simulink model "SupervisorFSM_RX"  (R2023b)
settings: Solver=FixedStepDiscrete  StartTime=0.0  StopTime=10.0  FixedStep=Ts_SupervisorFSM_RX  RelTol=1e-3  EnableMultiTasking=on
undefined symbols (not defined in the file): InitConfParams
settings Model: DataDictionary=EmbeddedBoardDD.sldd  Creator=vvasco  LastModifiedBy=upattacini
settings SolverCC: AllowMultiTaskInputOutput=on  AlgebraicLoopSolver=TrustRegion  AutoInsertRateTranBlk=on  InsertRTBMode=Never (minimum delay)
settings DataIOCC: LimitDataPoints=on  SaveOutput=off  SignalLogging=off  DSMLogging=off  SaveTime=off  ReturnWorkspaceOutputs=off
settings OptimizationCC: DefaultParameterBehavior=Inlined  DefaultUnderspecifiedDataType=single  StrengthReduction=on  PassReuseOutputArgsAs=Individual arguments  ZeroExternalMemoryAtStartup=off  ZeroInternalMemoryAtStartup=off  OptimizeBlockOrder=speed  OptimizationPriority=Speed  OptimizationCustomize=off  MultiThreadedLoops=on  EfficientTunableParamExpr=on
settings DebuggingCC: ParameterPrecisionLossMsg=none  UnconnectedInputMsg=warning  UnconnectedOutputMsg=warning  UnconnectedLineMsg=warning  AllowSymbolicDim=off  SFUnexpectedBacktrackingDiag=warning  SFNoUnconditionalDefaultTransitionDiag=warning  SFExecutionAtInitializationDiag=none  ArithmeticOperatorsInVariantConditions=warning
settings HardwareCC: ProdBitPerPointer=32  ProdBitPerSizeT=32  ProdBitPerPtrDiffT=32  ProdLargestAtomicInteger=Long  ProdLargestAtomicFloat=Double  ProdWordSize=32  ProdHWDeviceType=ARM Compatible->ARM Cortex-M
settings ModelReferenceCC: UpdateModelReferenceTargets=Force  EnableRefExpFcnMdlSchedulingChecks=on  ModelReferenceNumInstancesAllowed=Single
settings SFSimCC: SimUseLocalCustomCode=off  MATLABDynamicMemAlloc=off  CustomCodeUndefinedFunction=UseInterfaceOnly
settings SFSimCC: SimCustomHeaderCode=|
  | #include "rtw_enable_disable_motors.h"
  | #include "rtw_motor_config.h"
settings SFSimCC: SimUserSources=|
  | rtw_enable_disable_motors.c
  | rtw_motor_config.c
settings RTWCC: Description=Embedded Coder  SystemTargetFile=ert.tlc  GenCodeOnly=on  PackageGeneratedCodeAndArtifacts=on  PackageName=SupervisorFSM_RX  TemplateMakefile=ert_default_tmf  GenerateReport=on  RTWUseLocalCustomCode=off  RTWUseSimCustomCode=on  LaunchReport=on  TargetLang=C++  GenerateCodeReplacementReport=on  DLArmComputeVersion=19.05
settings RTWCC: CustomHeaderCode=|
  | #include "rtw_enable_disable_motors.h"
  | #include "rtw_motor_config.h"
settings RTWCC: CustomSource=|
  | rtw_enable_disable_motors.c
  | rtw_motor_config.c
settings CodeAppCC: ForceParamTrailComments=on  IgnoreCustomStorageClasses=off  MaxIdLength=60  OperatorAnnotations=on  SimulinkDataObjDesc=on  SFDataObjDesc=on  InsertBlockDesc=on
settings ERTTargetCC: TargetLangStandard=C++03 (ISO)  CodeReplacementLibrary=ARM Cortex-M,iCubTech  GenerateSampleERTMain=on  SupportVariableSizeSignals=on  InlinedParameterPlacement=NonHierarchical  RootIOFormat=Structure reference  ERTCustomFileTemplate=example_file_process.tlc
settings ConfigComp: CovMetricSettings=dw  CovSaveCumulativeToWorkspaceVar=on  CovSaveSingleToWorkspaceVar=on  CovExternalEMLEnable=off

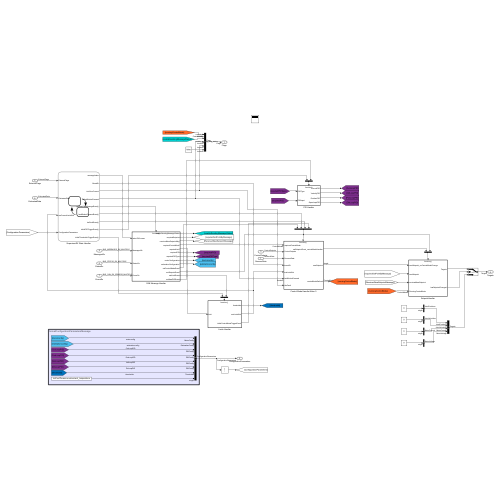
[thumbnail: Simulink's stored preview of the top-level diagram]
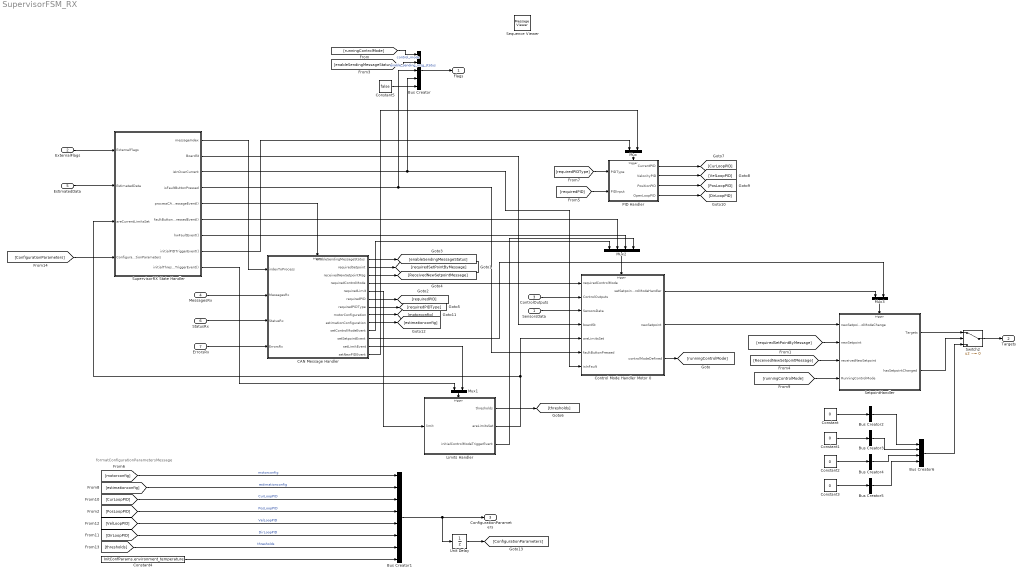
== system SupervisorFSM_RX ==
  note: formatConfigurationParametersMessage
  SensorsData : Inport  OutDataTypeStr=Bus: SensorsData  BusOutputAsStruct=on
  ExternalFlags : Inport  Port=2  OutDataTypeStr=Bus: ExternalFlags  BusOutputAsStruct=on
  ControlOutputs : Inport  Port=3  OutDataTypeStr=Bus: ControlOutputs  BusOutputAsStruct=on
  MessagesRx : Inport  Port=4  OutDataTypeStr=Bus: BUS_MESSAGES_RX_MULTIPLE  BusOutputAsStruct=on
  EstimatedData : Inport  Port=5  OutDataTypeStr=Bus: EstimatedData  BusOutputAsStruct=on
  StatusRx : Inport  Port=6  OutDataTypeStr=Bus: BUS_STATUS_RX_MULTIPLE  BusOutputAsStruct=on
  ErrorsRx : Inport  Port=7  OutDataTypeStr=Bus: BUS_CAN_RX_ERRORS_MULTIPLE  BusOutputAsStruct=on
  Bus Creator : BusCreator  Inputs=5  OutDataTypeStr=Bus: Flags  NonVirtualBus=on
      settings: InheritFromInputs=off
  Bus Creator1 : BusCreator  Inputs=8  OutDataTypeStr=Bus: ConfigurationParameters  NonVirtualBus=on
      settings: InheritFromInputs=off
  Bus Creator2 : BusCreator  Inputs=1  OutDataTypeStr=Bus: JointPositions  NonVirtualBus=on
      settings: InheritFromInputs=off
  Bus Creator3 : BusCreator  Inputs=1  OutDataTypeStr=Bus: JointVelocities  NonVirtualBus=on
      settings: InheritFromInputs=off
  Bus Creator4 : BusCreator  Inputs=1  OutDataTypeStr=Bus: MotorCurrent  NonVirtualBus=on
      settings: InheritFromInputs=off
  Bus Creator5 : BusCreator  Inputs=1  OutDataTypeStr=Bus: MotorVoltage  NonVirtualBus=on
      settings: InheritFromInputs=off
  Bus Creator6 : BusCreator  Inputs=4  OutDataTypeStr=Bus: Targets  NonVirtualBus=on
      settings: InheritFromInputs=off
  CAN Message Handler : Subsystem
  Constant{,1..3} (4 alike) : Constant  Value=0  OutDataTypeStr=single
  Constant4 : Constant  Value=InitConfParams.environment_temperature
  Constant5 : Constant  Value=false  OutDataTypeStr=boolean
  Control Mode Handler Motor 0 : Subsystem  TreatAsAtomicUnit=on
  Limits Handler : Subsystem  TreatAsAtomicUnit=on
  Mux : Mux  Inputs=2
  Mux1 : Mux  Inputs=2
  Mux2 : Mux
  Mux3 : Mux  Inputs=2
  PID Handler : Subsystem
  Sequence Viewer : MessageViewer  History=1000  SavedRootId=#
  SetpointHandler : Subsystem  TreatAsAtomicUnit=on
  SupervisorRX State Handler : Stateflow chart  TreatAsAtomicUnit=on
  Switch2 : Switch  Criteria=u2 ~= 0  SaturateOnIntegerOverflow=off  InputSameDT=off
  Unit Delay : UnitDelay  SampleTime=-1  HasFrameUpgradeWarning=on
  Flags : Outport  OutDataTypeStr=Bus: Flags  BusOutputAsStruct=on
  Targets : Outport  Port=2  OutDataTypeStr=Bus: Targets  BusOutputAsStruct=on
  ConfigurationParameters : Outport  Port=3  OutDataTypeStr=Bus: ConfigurationParameters  BusOutputAsStruct=on
  wires:
  ControlOutputs/1 -> Control Mode Handler Motor 0/2(ControlOutputs)
  ExternalFlags/1 -> SupervisorRX State Handler/1(ExternalFlags)
  SupervisorRX State Handler/1(messageIndex) -> CAN Message Handler/1(indexToProcess)
  SupervisorRX State Handler/2(BoardSt) -> Control Mode Handler Motor 0/4(boardSt)
  SupervisorRX State Handler/3(isInOverCurrent) -> Control Mode Handler Motor 0/7(isInFault), Bus Creator/4
  SupervisorRX State Handler/5(processCANMessageEvent()) -> CAN Message Handler/Trigger
  StatusRx/1 -> CAN Message Handler/3(StatusRx)
  MessagesRx/1 -> CAN Message Handler/2(MessagesRx)
  ErrorsRx/1 -> CAN Message Handler/4(ErrorsRx)
  CAN Message Handler/1(enableSendingMessageStatus) -> [enableSendingMessageStatus]
  CAN Message Handler/2(requiredSetpoint) -> [requiredSetPointByMessage]
  CAN Message Handler/4(requiredControlMode) -> Control Mode Handler Motor 0/1(requiredControlMode)
  CAN Message Handler/11(setSetpointEvent) -> Mux3/2
  CAN Message Handler/12(setLimitEvent) -> Mux1/2
  CAN Message Handler/5(requiredLimit) -> Limits Handler/1(limit)
  CAN Message Handler/10(setControlModeEvent) -> Mux2/1
  Limits Handler/1(thresholds) -> [thresholds]
  Limits Handler/2(areLimitsSet) -> Control Mode Handler Motor 0/5(areLimitsSet), SupervisorRX State Handler/3(areCurrentLimitsSet)
  SensorsData/1 -> Control Mode Handler Motor 0/3(SensorsData)
  SupervisorRX State Handler/4(isFaultButtonPressed) -> Control Mode Handler Motor 0/6(faultButtonPressed), Bus Creator/3
  Control Mode Handler Motor 0/1(setSetpointEvent_controlModeHandler) -> Mux3/1
  Control Mode Handler Motor 0/3(controlModeDefined) -> [runningControlMode]
  Control Mode Handler Motor 0/2(newSetpoint) -> SetpointHandler/1(newSetpoint_onControlModeChange)
  SupervisorRX State Handler/6(faultButtonPressedEvent()) -> Mux2/2
  SupervisorRX State Handler/7(hwFaultEvent()) -> Mux2/3
  Mux2/1 -> Control Mode Handler Motor 0/Trigger
  [runningControlMode] -> Bus Creator/1  "control_mode"
  [enableSendingMessageStatus] -> Bus Creator/2  "enable_sending_msg_status"
  Bus Creator/1 -> Flags/1
  [requiredSetPointByMessage] -> SetpointHandler/2(newSetpoint)
  SetpointHandler/2(hasSetpointChanged) -> Switch2/2
  Switch2/1 -> Targets/1
  SetpointHandler/1(Targets) -> Switch2/1
  Bus Creator2/1 -> Bus Creator6/1
  Constant3/1 -> Bus Creator5/1
  Bus Creator3/1 -> Bus Creator6/2
  Bus Creator5/1 -> Bus Creator6/4
  Bus Creator4/1 -> Bus Creator6/3
  Constant2/1 -> Bus Creator4/1
  Constant1/1 -> Bus Creator3/1
  Constant/1 -> Bus Creator2/1
  Bus Creator6/1 -> Switch2/3
  Bus Creator1/1 -> ConfigurationParameters/1, Unit Delay/1
  Mux3/1 -> SetpointHandler/Trigger
  CAN Message Handler/3(receivedNewSetpointMsg) -> [ReceivedNewSetpointMessage]
  [ReceivedNewSetpointMessage] -> SetpointHandler/3(receivedNewSetpoint)
  [runningControlMode] -> SetpointHandler/4(RunningControlMode)
  Limits Handler/3(initialControlModeTriggerEvent) -> Mux2/4
  CAN Message Handler/13(setNewPIDEvent) -> Mux/2
  CAN Message Handler/6(requiredPID) -> [requiredPID]
  CAN Message Handler/7(requiredPIDType) -> [requiredPIDType]
  [requiredPIDType] -> PID Handler/1(PIDType)
  [requiredPID] -> PID Handler/2(PIDInput)
  PID Handler/1(CurrentPID) -> [CurLoopPID]
  PID Handler/2(VelocityPID) -> [VelLoopPID]
  PID Handler/3(PositionPID) -> [PosLoopPID]
  PID Handler/4(OpenLoopPID) -> [DirLoopPID]
  CAN Message Handler/8(motorConfiguration) -> [motorconfig]
  CAN Message Handler/9(estimationConfiguration) -> [estimationconfig]
  [PosLoopPID] -> Bus Creator1/4  "PosLoopPID"
  [VelLoopPID] -> Bus Creator1/5  "VelLoopPID"
  [DirLoopPID] -> Bus Creator1/6  "DirLoopPID"
  [CurLoopPID] -> Bus Creator1/3  "CurLoopPID"
  [motorconfig] -> Bus Creator1/1  "motorconfig"
  [estimationconfig] -> Bus Creator1/2  "estimationconfig"
  [thresholds] -> Bus Creator1/7  "thresholds"
  Unit Delay/1 -> [ConfigurationParameters]
  [ConfigurationParameters] -> SupervisorRX State Handler/4(ConfigurationParameters)
  Mux/1 -> PID Handler/Trigger
  Mux1/1 -> Limits Handler/Trigger
  SupervisorRX State Handler/8(initialPIDTriggerEvent()) -> Mux/1
  SupervisorRX State Handler/9(initialThresholdsTriggerEvent()) -> Mux1/1
  EstimatedData/1 -> SupervisorRX State Handler/2(EstimatedData)
  Constant4/1 -> Bus Creator1/8
  Constant5/1 -> Bus Creator/5

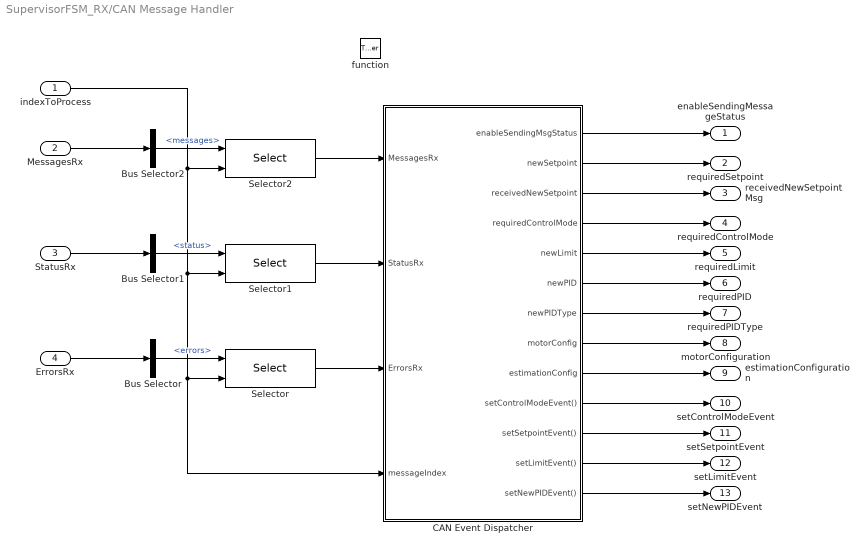
== system SupervisorFSM_RX/CAN Message Handler ==
  indexToProcess : Inport
  MessagesRx : Inport  Port=2  OutDataTypeStr=Bus: BUS_MESSAGES_RX_MULTIPLE
  StatusRx : Inport  Port=3  OutDataTypeStr=Bus: BUS_STATUS_RX_MULTIPLE
  ErrorsRx : Inport  Port=4  OutDataTypeStr=Bus: BUS_CAN_RX_ERRORS_MULTIPLE
  function : TriggerPort  TriggerType=function-call  VariantControl=(inherit)
  Bus Selector : BusSelector  OutputSignals=errors
  Bus Selector1 : BusSelector  OutputSignals=status
  Bus Selector2 : BusSelector  OutputSignals=messages
  CAN Event Dispatcher : Stateflow chart  TreatAsAtomicUnit=on
      settings: PortSchema="{\"entries\":[{\"content\":{\"sides\":[{\"content\":{\"connectorIds\":[\"In3\",\"In2\",\"In1\",\"In4\"]},\"type\":\"ConnectorPlacement.EquallySpacedRectSide\",\"uuid\":\"262d8322-eee9-4d2f-8394-9ad0f57315f2\"},{\"content\":{\"connectorIds\":[\"Out4\",\"Out2\",\"Out5\",\"Out1\",\"Out3\",\"Out6\",\"Out7\",\"Out8\",\"Out9\",\"Out10\",\"Out11\",\"Out12\",\"Out13\"],\"side\":\"RIGHT\"},\"type\":\"ConnectorPlacement.EquallySpacedRectSide\",\"uuid\":\"ca9d82ac-748f-4018-bf9f-4633821aba3f\"},{\"content\":{\"connectorIds\":[],\"side\":\"TOP\"},\"type\":\"ConnectorPlacement.EquallySpacedRectSide\",\"uuid\":\"6799758e-9858-4ae3-a4b1-29346dfc98be\"}]},\"type\":\"ConnectorPlacement.EquallySpacedConnector\",\"uuid\":\"ac16e6b5-85f8-470c-98ca-7de9ad02246e\"}],\"packageUris\":[\"http://schema.mathworks.com/mf0/Connector/R2020b\"],\"version\":\"1.0\"}"
  Selector : Selector  NumberOfDimensions=2  InputPortWidth=3  IndexOptions=Index vector (dialog),Index vector (port)  Indices=1,1  OutputSizes=1,1
  Selector1 : Selector  NumberOfDimensions=2  InputPortWidth=3  IndexOptions=Index vector (dialog),Index vector (port)  Indices=1,1  OutputSizes=1,1
  Selector2 : Selector  NumberOfDimensions=2  InputPortWidth=3  IndexOptions=Index vector (dialog),Index vector (port)  Indices=1,1  OutputSizes=1,1
  enableSendingMessageStatus : Outport
  requiredSetpoint : Outport  Port=2
  receivedNewSetpointMsg : Outport  Port=3
  requiredControlMode : Outport  Port=4
  requiredLimit : Outport  Port=5
  requiredPID : Outport  Port=6  OutDataTypeStr=Bus: BUS_MSG_PID
  requiredPIDType : Outport  Port=7
  motorConfiguration : Outport  Port=8  OutDataTypeStr=Bus: MotorConfig
  estimationConfiguration : Outport  Port=9  OutDataTypeStr=Bus: EstimationConfig
  setControlModeEvent : Outport  Port=10
  setSetpointEvent : Outport  Port=11
  setLimitEvent : Outport  Port=12
  setNewPIDEvent : Outport  Port=13
  wires:
  ErrorsRx/1 -> Bus Selector/1
  StatusRx/1 -> Bus Selector1/1
  MessagesRx/1 -> Bus Selector2/1
  Bus Selector2/1 -> Selector2/1  "<messages>"
  Bus Selector1/1 -> Selector1/1  "<status>"
  Bus Selector/1 -> Selector/1  "<errors>"
  indexToProcess/1 -> Selector1/2, CAN Event Dispatcher/4(messageIndex), Selector/2, Selector2/2
  Selector/1 -> CAN Event Dispatcher/1(ErrorsRx)
  Selector1/1 -> CAN Event Dispatcher/2(StatusRx)
  Selector2/1 -> CAN Event Dispatcher/3(MessagesRx)
  CAN Event Dispatcher/1(requiredControlMode) -> requiredControlMode/1
  CAN Event Dispatcher/10(setControlModeEvent()) -> setControlModeEvent/1
  CAN Event Dispatcher/11(setSetpointEvent()) -> setSetpointEvent/1
  CAN Event Dispatcher/12(setLimitEvent()) -> setLimitEvent/1
  CAN Event Dispatcher/4(enableSendingMsgStatus) -> enableSendingMessageStatus/1
  CAN Event Dispatcher/2(newSetpoint) -> requiredSetpoint/1
  CAN Event Dispatcher/3(newLimit) -> requiredLimit/1
  CAN Event Dispatcher/5(receivedNewSetpoint) -> receivedNewSetpointMsg/1
  CAN Event Dispatcher/6(newPID) -> requiredPID/1
  CAN Event Dispatcher/7(newPIDType) -> requiredPIDType/1
  CAN Event Dispatcher/8(motorConfig) -> motorConfiguration/1
  CAN Event Dispatcher/13(setNewPIDEvent()) -> setNewPIDEvent/1
  CAN Event Dispatcher/9(estimationConfig) -> estimationConfiguration/1

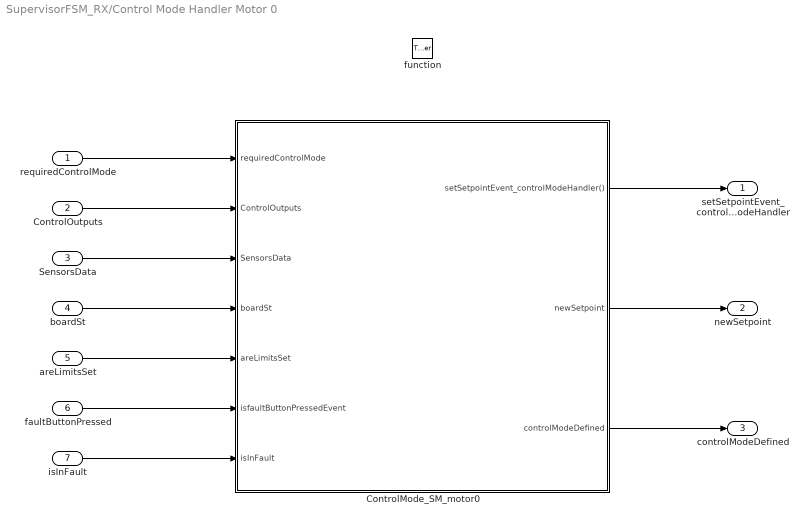
== system SupervisorFSM_RX/Control Mode Handler Motor 0 ==
  requiredControlMode : Inport  OutDataTypeStr=Enum: ControlModes
  ControlOutputs : Inport  Port=2  OutDataTypeStr=Bus: ControlOutputs
  SensorsData : Inport  Port=3  OutDataTypeStr=Bus: SensorsData
  boardSt : Inport  Port=4
  areLimitsSet : Inport  Port=5
  faultButtonPressed : Inport  Port=6  OutDataTypeStr=boolean
  isInFault : Inport  Port=7
  function : TriggerPort  TriggerType=function-call  VariantControl=(inherit)  OutputDataType=double
  ControlMode_SM_motor0 : Stateflow chart  TreatAsAtomicUnit=on
      settings: PortSchema="{\"entries\":[{\"content\":{\"sides\":[{\"content\":{\"connectorIds\":[\"In3\",\"In5\",\"In4\",\"In1\",\"In2\",\"In6\",\"In7\"]},\"type\":\"ConnectorPlacement.EquallySpacedRectSide\",\"uuid\":\"16512c25-bd76-4850-9767-5b856cef53aa\"},{\"content\":{\"connectorIds\":[\"Out3\",\"Out1\",\"Out2\"],\"side\":\"RIGHT\"},\"type\":\"ConnectorPlacement.EquallySpacedRectSide\",\"uuid\":\"18a45251-a2e9-43d4-bd88-b12ad9528921\"},{\"content\":{\"connectorIds\":[],\"side\":\"TOP\"},\"type\":\"ConnectorPlacement.EquallySpacedRectSide\",\"uuid\":\"fd5907c5-7215-4be4-b0f8-eb015da6c502\"}]},\"type\":\"ConnectorPlacement.EquallySpacedConnector\",\"uuid\":\"dd0cc5ef-a33e-40fc-9b84-b3bdf02167fe\"}],\"packageUris\":[\"http://schema.mathworks.com/mf0/Connector/R2020b\"],\"version\":\"1.0\"}"
  setSetpointEvent_controlModeHandler : Outport
  newSetpoint : Outport  Port=2  OutDataTypeStr=single
  controlModeDefined : Outport  Port=3  OutDataTypeStr=Enum: ControlModes
  wires:
  boardSt/1 -> ControlMode_SM_motor0/1(boardSt)
  areLimitsSet/1 -> ControlMode_SM_motor0/2(areLimitsSet)
  requiredControlMode/1 -> ControlMode_SM_motor0/3(requiredControlMode)
  SensorsData/1 -> ControlMode_SM_motor0/4(SensorsData)
  ControlOutputs/1 -> ControlMode_SM_motor0/5(ControlOutputs)
  ControlMode_SM_motor0/2(controlModeDefined) -> controlModeDefined/1
  ControlMode_SM_motor0/1(newSetpoint) -> newSetpoint/1
  ControlMode_SM_motor0/3(setSetpointEvent_controlModeHandler()) -> setSetpointEvent_controlModeHandler/1
  faultButtonPressed/1 -> ControlMode_SM_motor0/6(isfaultButtonPressedEvent)
  isInFault/1 -> ControlMode_SM_motor0/7(isInFault)

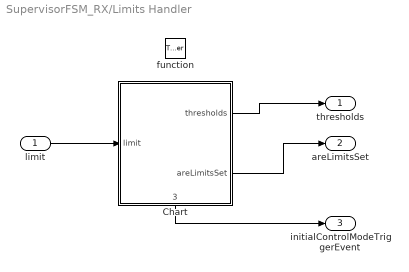
== system SupervisorFSM_RX/Limits Handler ==
  limit : Inport
  function : TriggerPort  TriggerType=function-call  VariantControl=(inherit)
  Chart : Stateflow chart  TreatAsAtomicUnit=on
      settings: PortSchema="{\"entries\":[{\"content\":{\"sides\":[{\"content\":{\"connectorIds\":[\"In1\"]},\"type\":\"ConnectorPlacement.EquallySpacedRectSide\",\"uuid\":\"0584a8d9-54fc-4826-bb82-8ee436931ccb\"},{\"content\":{\"connectorIds\":[\"Out1\",\"Out2\"],\"side\":\"RIGHT\"},\"type\":\"ConnectorPlacement.EquallySpacedRectSide\",\"uuid\":\"1e00f1d2-76af-45ba-9501-0555e9c73a7d\"},{\"content\":{\"connectorIds\":[],\"side\":\"TOP\"},\"type\":\"ConnectorPlacement.EquallySpacedRectSide\",\"uuid\":\"c8be2aa1-781d-4a54-8da4-289e5dceeb67\"},{\"content\":{\"connectorIds\":[\"Out3\"],\"side\":\"BOTTOM\"},\"type\":\"ConnectorPlacement.EquallySpacedRectSide\",\"uuid\":\"c0009a38-640d-457e-891e-a241b21e5d3e\"}]},\"type\":\"ConnectorPlacement.EquallySpacedConnector\",\"uuid\":\"a709c32b-ef0c-4b14-b7ff-ec32eaa315cd\"}],\"packageUris\":[\"http://schema.mathworks.com/mf0/Connector/R2020b\"],\"version\":\"1.0\"}"
  thresholds : Outport
  areLimitsSet : Outport  Port=2
  initialControlModeTriggerEvent : Outport  Port=3
  wires:
  Chart/1(thresholds) -> thresholds/1
  Chart/2(areLimitsSet) -> areLimitsSet/1
  limit/1 -> Chart/1(limit)
  Chart/3(initialControlModeTriggerEvent()) -> initialControlModeTriggerEvent/1

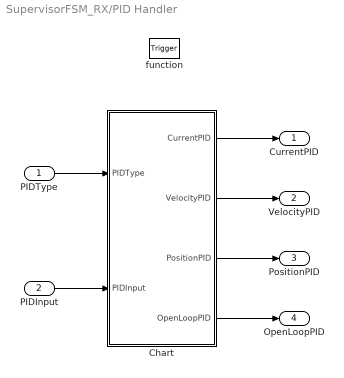
== system SupervisorFSM_RX/PID Handler ==
  PIDType : Inport
  PIDInput : Inport  Port=2
  function : TriggerPort  TriggerType=function-call  VariantControl=(inherit)
  Chart : Stateflow chart  TreatAsAtomicUnit=on
  CurrentPID : Outport
  VelocityPID : Outport  Port=2
  PositionPID : Outport  Port=3
  OpenLoopPID : Outport  Port=4
  wires:
  PIDType/1 -> Chart/1(PIDType)
  PIDInput/1 -> Chart/2(PIDInput)
  Chart/2(VelocityPID) -> VelocityPID/1
  Chart/3(PositionPID) -> PositionPID/1
  Chart/4(OpenLoopPID) -> OpenLoopPID/1
  Chart/1(CurrentPID) -> CurrentPID/1

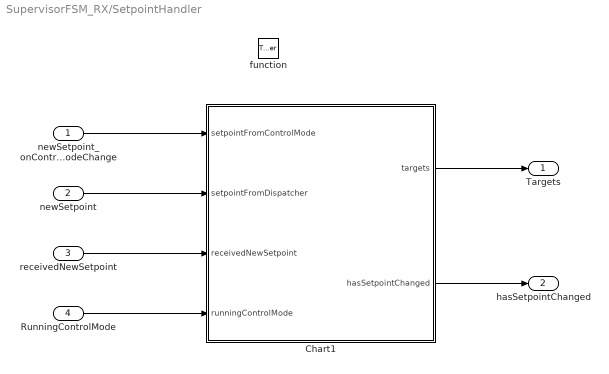
== system SupervisorFSM_RX/SetpointHandler ==
  newSetpoint_onControlModeChange : Inport
  newSetpoint : Inport  Port=2
  receivedNewSetpoint : Inport  Port=3
  RunningControlMode : Inport  Port=4  OutDataTypeStr=Enum: ControlModes
  function : TriggerPort  TriggerType=function-call  VariantControl=(inherit)
  Chart1 : Stateflow chart  TreatAsAtomicUnit=on
  Targets : Outport  OutDataTypeStr=Bus: Targets
  hasSetpointChanged : Outport  Port=2
  wires:
  newSetpoint_onControlModeChange/1 -> Chart1/1(setpointFromControlMode)
  newSetpoint/1 -> Chart1/2(setpointFromDispatcher)
  Chart1/2(hasSetpointChanged) -> hasSetpointChanged/1
  Chart1/1(targets) -> Targets/1
  receivedNewSetpoint/1 -> Chart1/3(receivedNewSetpoint)
  RunningControlMode/1 -> Chart1/4(runningControlMode)

== stateflow chart SupervisorFSM_RX/Limits Handler/Chart ==
  state Home
  (junction 31) -> (junction 33)
  (junction 11) -> (junction 31) [order 1] : [areLimitsSet == false]
      | {areLimitsSet = true;
      | send(initialControlModeTriggerEvent);}
  (junction 33) -> (junction 21)
  (junction 11) -> (junction 21) [order 2]
  (junction 2) -> (junction 11) [order 1] : [limit.type == ControlModes.Current]
      | {thresholds.motorNominalCurrents = abs(limit.nominal);
      | thresholds.motorPeakCurrents = abs(limit.peak);
      | thresholds.motorOverloadCurrents = abs(limit.overload);}
  (junction 21) -> Home
  (default) -> (junction 2) : {thresholds=InitConfParams.thresholds;}
  Home -> (junction 2)
  (junction 2) -> (junction 16) [order 2]
  (junction 25) -> Home
  (junction 16) -> (junction 25)
  data: thresholds output Bus: Thresholds; areLimitsSet output boolean =false; limit input Bus: SV_Limits; InitConfParams parameter Bus: ConfigurationParameters
  events: initialControlModeTriggerEvent output FUNCTION_CALL_EVENT

== stateflow chart SupervisorFSM_RX/SupervisorRX State Handler ==
  state STATE_HANDLER [parallel]
    settings: executionOrder=1
    note: ATTENTION :
        | Currently the events "BoardFaultEvent" and "OutOfBoardFaultEvent"
        | are not sent by any state. They are simple placeholder.
    state NotConfigured
      entry:
      BoardSt = BoardState.NotConfigured;
    state Fault
      entry:
      BoardSt = BoardState.Fault;
    state Configured
      entry:
      BoardSt = BoardState.Configured;
    (default) -> NotConfigured
    NotConfigured -> Fault [order 1] : BoardFaultEvent
    (junction 548) -> NotConfigured [order 1] : [!isBoardConfigured()]
    NotConfigured -> Configured [order 2] : [isBoardConfigured()]
    (junction 548) -> Configured [order 2]
    Fault -> (junction 548) : OutOfBoardFaultEvent
    Configured -> Fault : BoardFaultEvent
  state FAULT_HANDLER [parallel]
    settings: executionOrder=2
    state FaultButtonPressed [parallel]
      settings: executionOrder=1
      state NoFault
        entry:
        isFaultButtonPressed = false;
      state ButtonPressed
        entry:
        isFaultButtonPressed = true;
        send(faultButtonPressedEvent);
      (default) -> FAULT_HANDLER.FaultButtonPressed.NoFault
      ButtonPressed -> FAULT_HANDLER.FaultButtonPressed.NoFault : [hasChangedTo(ExternalFlags.fault_button, false)]
      FAULT_HANDLER.FaultButtonPressed.NoFault -> ButtonPressed : [hasChangedTo(ExternalFlags.fault_button, true)]
    state OverCurrent [parallel]
      settings: executionOrder=2
      state NoFault
        entry:
        isInOverCurrent=false;
      state LimitNonConfigured
      state OverCurrentFault
        entry:
        isInOverCurrent=true;
        send(hwFaultEvent);
      (default) -> LimitNonConfigured
      LimitNonConfigured -> FAULT_HANDLER.OverCurrent.NoFault : [areCurrentLimitsSet==true]
      FAULT_HANDLER.OverCurrent.NoFault -> OverCurrentFault : [abs(EstimatedData.Iq_filtered.current) >= ConfigurationParameters.thresholds.motorOverloadCurrents]
      OverCurrentFault -> FAULT_HANDLER.OverCurrent.NoFault : [abs(EstimatedData.Iq_filtered.current) < ConfigurationParameters.thresholds.motorOverloadCurrents]
  state CAN_MESSAGES_FOR_LOOP [parallel]
    settings: executionOrder=3
    state state1
    (default) -> (junction 514) : {send(initialPIDTriggerEvent);
        | send(initialThresholdsTriggerEvent);}
    (junction 513) -> (junction 514)
    (junction 519) -> (junction 513)
    (junction 514) -> (junction 516) : {messageIndex = 1;}
    (junction 516) -> (junction 515) [order 1] : [messageIndex <= CAN_MAX_NUM_PACKETS]
    (junction 515) -> (junction 517) : {send(processCANMessageEvent);}
    (junction 518) -> (junction 516)
    (junction 516) -> state1 [order 2]
    (junction 517) -> (junction 518) : {messageIndex = messageIndex + 1;}
    state1 -> (junction 519)
  data: boardOk function_output boolean; ExternalFlags input Bus: ExternalFlags; EstimatedData input Bus: EstimatedData; areCurrentLimitsSet input boolean; messageIndex output int32; BoardSt output Enum: BoardState =BoardState.NotConfigured; isInOverCurrent output boolean =false; isFaultButtonPressed output boolean =false; ConfigurationParameters input Bus: ConfigurationParameters; CAN_MAX_NUM_PACKETS parameter
  events: BoardFaultEvent local FUNCTION_CALL_EVENT; OutOfBoardFaultEvent local FUNCTION_CALL_EVENT; processCANMessageEvent output FUNCTION_CALL_EVENT; faultButtonPressedEvent output FUNCTION_CALL_EVENT; hwFaultEvent output FUNCTION_CALL_EVENT; initialPIDTriggerEvent output FUNCTION_CALL_EVENT; initialThresholdsTriggerEvent output FUNCTION_CALL_EVENT
  function boardOk=isBoardConfigured:
    | function boardOk=isBoardConfigured
    | %check here if all board services are ready 
    | boardOk=true;
    | end

== stateflow chart SupervisorFSM_RX/PID Handler/Chart ==
  state home
  (default) -> (junction 7)
  (junction 7) -> (junction 9) : {PositionPID = InitConfParams.PosLoopPID;
      | CurrentPID = InitConfParams.CurLoopPID;
      | VelocityPID = InitConfParams.VelLoopPID;}
  (junction 9) -> (junction 17) [order 5]
  (junction 34) -> (junction 9)
  (junction 9) -> (junction 37) [order 4] : [PIDType == ControlModes.Velocity]
  (junction 9) -> (junction 15) [order 3] : [PIDType == ControlModes.Voltage]
  (junction 9) -> (junction 11) [order 1] : [PIDType == ControlModes.Current]
  (junction 17) -> (junction 27)
  (junction 32) -> (junction 34)
  (junction 9) -> (junction 13) [order 2] : [PIDType == ControlModes.Position]
  (junction 11) -> (junction 19) : {CurrentPID.P = PIDInput.Kp;
      | CurrentPID.I = PIDInput.Ki;
      | CurrentPID.D = PIDInput.Kd;
      | CurrentPID.shift_factor = PIDInput.Ks;}
  (junction 13) -> home : {PositionPID.P = PIDInput.Kp;
      | PositionPID.I = PIDInput.Ki;
      | PositionPID.D = PIDInput.Kd;
      | PositionPID.shift_factor = PIDInput.Ks;}
  (junction 15) -> (junction 24) : {OpenLoopPID.P = PIDInput.Kp;
      | OpenLoopPID.I = PIDInput.Ki;
      | OpenLoopPID.D = PIDInput.Kd;
      | OpenLoopPID.shift_factor = PIDInput.Ks;}
  (junction 37) -> (junction 39) : {VelocityPID.P = PIDInput.Kp;
      | VelocityPID.I = PIDInput.Ki;
      | VelocityPID.D = PIDInput.Kd;
      | VelocityPID.shift_factor = PIDInput.Ks;}
  (junction 27) -> (junction 39)
  (junction 39) -> (junction 24)
  (junction 19) -> home
  (junction 24) -> home
  home -> (junction 30)
  (junction 30) -> (junction 32)
  data: PIDType input Enum: ControlModes; PIDInput input Bus: BUS_MSG_PID; CurrentPID output Bus: PIDConfig; VelocityPID output Bus: PIDConfig; PositionPID output Bus: PIDConfig; OpenLoopPID output Bus: PIDConfig; InitConfParams parameter Bus: ConfigurationParameters

== stateflow chart SupervisorFSM_RX/SetpointHandler/Chart1 ==
  note: The idea here is : first of all reset all the targets and then set only the value of the given setpoint. If we are in idel or HW fault all targets remain equal to 0.
  state init
  (junction 54) -> (junction 75) [order 1] : [CheckSetPointVoltage()]{newSetpoint = setpointFromDispatcher.voltage;}
  (junction 75) -> (junction 77)
  (default) -> (junction 8)
  (junction 54) -> (junction 77) [order 2] : [CheckSetPointCurrent()]{newSetpoint = setpointFromDispatcher.current;}
  (junction 77) -> (junction 79)
  (junction 8) -> (junction 54) [order 1] : [receivedNewSetpoint==true]
  (junction 9) -> (junction 8)
  (junction 54) -> (junction 79) [order 3] : [CheckSetPointVelocity()]{newSetpoint = setpointFromDispatcher.velocity;}
  (junction 54) -> (junction 81) [order 4] : {newSetpoint = 0;}
  (junction 8) -> (junction 59) [order 2] : {newSetpoint=setpointFromControlMode}
  (junction 22) -> (junction 9)
  (junction 79) -> (junction 81)
  (junction 81) -> (junction 59)
  (junction 59) -> (junction 6) : {targets.motorvoltage.voltage = 0;
      | targets.motorcurrent.current = 0;
      | targets.jointvelocities.velocity =0;
      | targets.jointpositions.position = 0;}
  (junction 6) -> (junction 11) [order 5]
  (junction 6) -> (junction 28) [order 4] : [CheckSetPointPosition()]
  (junction 6) -> (junction 19) [order 2] : [CheckSetPointVoltage()]
  (junction 6) -> (junction 18) [order 3] : [CheckSetPointVelocity()]
  (junction 6) -> (junction 20) [order 1] : [CheckSetPointCurrent()]
  (junction 11) -> (junction 32)
  (junction 18) -> (junction 14) : {targets.jointvelocities.velocity = newSetpoint;}
  (junction 28) -> (junction 16) : {targets.jointpositions.position = newSetpoint;}
  (junction 19) -> (junction 31) : {targets.motorvoltage.voltage = newSetpoint;}
  (junction 20) -> (junction 24) : {targets.motorcurrent.current = newSetpoint;}
  (junction 16) -> (junction 14)
  (junction 14) -> (junction 15)
  (junction 31) -> (junction 24)
  (junction 24) -> (junction 15)
  (junction 15) -> init : {hasSetpointChanged = true;}
  init -> (junction 22)
  (junction 32) -> init
  data: out function_output boolean size=1; out function_output boolean size=1; out function_output boolean size=1; out function_output boolean size=1; setpointFromControlMode input single; setpointFromDispatcher input Bus: BUS_MSG_DESIRED_TARGETS; targets output Bus: Targets; hasSetpointChanged output boolean =false; newSetpoint local single size=1; receivedNewSetpoint input boolean; runningControlMode input Enum: ControlModes
  function out = CheckSetPointCurrent:
    | function out = CheckSetPointCurrent
    |  
    | if (runningControlMode ==ControlModes.Current )
    |     out = true;
    | else 
    |     out = false;
    | end
  function out = CheckSetPointVoltage:
    | function out = CheckSetPointVoltage
    |  
    | if (runningControlMode ==ControlModes.Voltage )
    |     out = true;
    | else 
    |     out = false;
    | end
  function out = CheckSetPointPosition:
    | function out = CheckSetPointPosition
    |  
    | if (runningControlMode ==ControlModes.Position )
    |     out = true;
    | else 
    |     out = false;
    | end
  function out = CheckSetPointVelocity:
    | function out = CheckSetPointVelocity
    |  
    | if (runningControlMode ==ControlModes.Velocity )
    |     out = true;
    | else 
    |     out = false;
    | end

== stateflow chart SupervisorFSM_RX/CAN Message Handler/CAN Event Dispatcher ==
  state EVENT_DISPATCHER
    state Home
    (default) -> (junction 66) : {motorConfig=InitConfParams.motorconfig;
        | estimationConfig = InitConfParams.estimationconfig;}
    (junction 87) -> (junction 66)
    (junction 66) -> (junction 69) [order 2]
    (junction 85) -> (junction 87)
    (junction 69) -> (junction 71)
    (junction 66) -> (junction 42) [order 1] : [ErrorsRx.event==false]
    (junction 42) -> (junction 111) [order 5] : [StatusRx.motor_config==true]{formatMotorConfig(); hardwareConfigMotor()}
    (junction 42) -> (junction 105) [order 4] : [StatusRx.velocity_pid==true]
        | {newPIDType = ControlModes.Velocity;
        | newPID = MessagesRx.pid;
        | send(setNewPIDEvent);}
    (junction 42) -> (junction 143) [order 6] : [StatusRx.desired_targets == true]
        | {newSetpoint = MessagesRx.desired_targets;
        | enableSendingMsgStatus = true;
        | receivedNewSetpoint = true;
        | send(setSetpointEvent);}
    (junction 42) -> (junction 50) [order 3] : [StatusRx.current_pid==true]
        | {newPIDType = ControlModes.Current;
        | newPID = MessagesRx.pid;
        | send(setNewPIDEvent);}
    (junction 42) -> (junction 48) [order 2] : [StatusRx.current_limit==true]
        | {newLimit.type = ControlModes.Current;
        | newLimit.peak = MessagesRx.current_limit.peak;
        | newLimit.nominal = MessagesRx.current_limit.nominal;
        | newLimit.overload = MessagesRx.current_limit.overload;
        | send(setLimitEvent);}
    (junction 42) -> (junction 46) [order 1] : [StatusRx.control_mode==true]
        | {requiredControlMode = convert(MessagesRx.control_mode.mode); receivedNewSetpoint=false; send(setControlModeEvent);}
    (junction 42) -> (junction 90) [order 7]
    (junction 143) -> (junction 54)
    (junction 46) -> (junction 57)
    (junction 90) -> Home
    (junction 48) -> (junction 60)
    (junction 50) -> (junction 63)
    (junction 105) -> (junction 107)
    (junction 111) -> (junction 113)
    (junction 71) -> (junction 54)
    (junction 54) -> (junction 57)
    (junction 57) -> Home
    (junction 60) -> Home
    (junction 63) -> (junction 60)
    (junction 107) -> (junction 63)
    (junction 113) -> (junction 107)
    Home -> (junction 83)
    (junction 83) -> (junction 85) [order 1] : [messageIndex == 1]{enableSendingMsgStatus = false;}
    (junction 98) -> (junction 85)
    (junction 83) -> (junction 96) [order 2]
    (junction 96) -> (junction 98)
  data: controlmode function_output Enum: ControlModes size=1; mccontrolmode function_input Enum: MCControlModes size=1; ErrorsRx input Bus: BUS_CAN_RX_ERRORS; StatusRx input Bus: BUS_STATUS_RX; MessagesRx input Bus: BUS_MESSAGES_RX; requiredControlMode output Enum: ControlModes; newSetpoint output Bus: BUS_MSG_DESIRED_TARGETS; newLimit output Bus: SV_Limits; enableSendingMsgStatus output boolean; receivedNewSetpoint output boolean =false; InitConfParams parameter Bus: ConfigurationParameters; messageIndex input int32; newPID output Bus: BUS_MSG_PID; newPIDType output Enum: ControlModes; motorConfig output Bus: MotorConfig; estimationConfig output Bus: EstimationConfig
  events: setControlModeEvent output FUNCTION_CALL_EVENT; setSetpointEvent output FUNCTION_CALL_EVENT; setLimitEvent output FUNCTION_CALL_EVENT; setNewPIDEvent output FUNCTION_CALL_EVENT
  function formatMotorConfig:
    | function formatMotorConfig
    |     %#ok<*STRNU>
    |     motorConfig.use_index = MessagesRx.motor_config.use_index;
    |     motorConfig.pole_pairs = MessagesRx.motor_config.number_poles / 2;
    |     motorConfig.encoder_tolerance = MessagesRx.motor_config.encoder_tolerance;
    |     motorConfig.rotor_encoder_resolution = MessagesRx.motor_config.rotor_encoder_resolution;
    |     motorConfig.rotor_index_offset = MessagesRx.motor_config.rotor_index_offset;
    |     motorConfig.has_quadrature_encoder = MessagesRx.motor_config.has_quadrature_encoder;
    |     motorConfig.has_hall_sens = MessagesRx.motor_config.has_hall_sens;
    |     motorConfig.has_speed_quadrature_encoder = MessagesRx.motor_config.has_speed_quadrature_encoder;
    |     motorConfig.has_torque_sens = MessagesRx.motor_config.has_torque_sens;
    |     motorConfig.enable_verbosity = MessagesRx.motor_config.enable_verbosity; 
    | end
  function hardwareConfigMotor:
    | function hardwareConfigMotor
    |     swapBC = uint8(1);
    |     hall_sens_offset = uint16(motorConfig.hall_sens_offset*65536/360);
    |     
    |     rtw_configMotor(cast(motorConfig.has_quadrature_encoder, 'uint8'),...
    |                     motorConfig.rotor_encoder_resolution, ...
    |                     motorConfig.pole_pairs, ...
    |                     cast(motorConfig.has_hall_sens,'uint8'), ...
    |                     swapBC, hall_sens_offset);
    | end
  function controlmode = convert(mccontrolmode):
    | function controlmode = convert(mccontrolmode)
    | 
    |     if mccontrolmode == MCControlModes.Idle
    |         controlmode = ControlModes.Idle;
    |     elseif mccontrolmode == MCControlModes.Current
    |         controlmode = ControlModes.Current;
    |     elseif mccontrolmode == MCControlModes.SpeedVoltage
    |         controlmode = ControlModes.Velocity;
    |     elseif mccontrolmode == MCControlModes.OpenLoop
    |         controlmode = ControlModes.Voltage;
    |     else
    |         controlmode = ControlModes.Idle;
    |     end
    | 
    | end

== stateflow chart SupervisorFSM_RX/Control Mode Handler Motor 0/ControlMode_SM_motor0 ==
  state Torque [commented out]
  state NotConfigured
    entry:
    controlModeDefined = ControlModes.NotConfigured;
    rtw_disableMotor();
  state Idle
    entry:
    controlModeDefined = ControlModes.Idle;
    rtw_disableMotor();
    //this updates the targets value
    send(setSetpointEvent_controlModeHandler);
  state Position
    entry:
    controlModeDefined = ControlModes.Position;
    newSetpoint=SensorsData.jointpositions.position;
    send(setSetpointEvent_controlModeHandler);
  state Current
    entry:
    controlModeDefined = ControlModes.Current;
    send(setSetpointEvent_controlModeHandler);
  state HWFault
    entry:
    controlModeDefined = ControlModes.HwFaultCM;
    rtw_disableMotor();
    //this updates the targets value
    send(setSetpointEvent_controlModeHandler);
  state Voltage
    entry:
    controlModeDefined = ControlModes.Voltage;
    send(setSetpointEvent_controlModeHandler);
  note: IMPORTANT:
      | Currently we use IDLE command to exit from HWFault state,
      | but We should use FORCE_IDLE command when it will be implemented
  state Velocity
    entry:
    controlModeDefined = ControlModes.Velocity;
    newSetpoint=0;
    send(setSetpointEvent_controlModeHandler);
  (junction 353) -> (junction 355)
  (junction 350) -> (junction 353) [order 1] : [IsBoardReady() && isConfigurationSet()]
  (junction 355) -> (junction 214)
  (default) -> (junction 350)
  (junction 350) -> NotConfigured [order 2]
  NotConfigured -> (junction 213) [order 1] : [IsBoardReady() && isConfigurationSet()]
  (junction 213) -> (junction 214)
  (junction 211) -> (junction 214)
  (junction 329) -> (junction 213)
  (junction 214) -> Idle
  (junction 241) -> (junction 211)
  HWFault -> NotConfigured [order 1] : [!isInFault && IsNewCtrl_Idle() && !isConfigurationSet()]
  NotConfigured -> HWFault [order 2] : [isInFault]
  (junction 212) -> Idle
  (junction 220) -> (junction 212)
  Idle -> (junction 215) [order 2]
  (junction 215) -> Idle [order 2]
  (junction 215) -> (junction 221) [order 1] : [!IsNewCtrl_Idle()]{rtw_enableMotor();}
  (junction 216) -> Idle : [IsNewCtrl_Idle()]
  (junction 224) -> (junction 216) [order 2]
  (junction 217) -> Idle : [IsNewCtrl_Idle()]
  (junction 223) -> (junction 217) [order 2]
  (junction 218) -> Idle : [IsNewCtrl_Idle()]
  (junction 226) -> (junction 218) [order 2]
  Idle -> (junction 222) [order 1] : [isInFault || isfaultButtonPressedEvent]
  (junction 222) -> (junction 219)
  (junction 219) -> (junction 229)
  Position -> (junction 220) [order 3] : [IsNewCtrl_Idle()]
  (junction 221) -> Position [order 1] : [IsNewCtrl_Position()]
  (junction 221) -> (junction 227) [order 2]
  (junction 224) -> Position [order 1] : [IsNewCtrl_Position()]
  (junction 331) -> (junction 224) [order 1] : [!IsNewCtrl_Current()]
  Position -> (junction 225) [order 2] : [!IsNewCtrl_Idle()]
  (junction 225) -> (junction 332) : [!IsNewCtrl_Position()]
  (junction 223) -> Position [order 1] : [IsNewCtrl_Position()]
  (junction 335) -> (junction 223) [order 2]
  (junction 226) -> Position [order 1] : [IsNewCtrl_Position()]
  (junction 338) -> (junction 226) [order 2]
  Position -> (junction 228) [order 1] : [isInFault || isfaultButtonPressedEvent]
  (junction 228) -> (junction 229)
  (junction 229) -> (junction 330)
  (junction 227) -> Current [order 1] : [IsNewCtrl_Current()]{ newSetpoint=0; }
  (junction 331) -> Current [order 2]
  (junction 227) -> (junction 339) [order 2]
  Current -> (junction 331) [order 3]
  (junction 332) -> (junction 333) [order 1] : [IsNewCtrl_Current()]
  (junction 333) -> Current : {newSetpoint=ControlOutputs.Iq_fbk.current;}
  (junction 332) -> (junction 341) [order 2]
  (junction 335) -> (junction 334) [order 1] : [IsNewCtrl_Current()]
  (junction 334) -> (junction 337)
  (junction 343) -> (junction 335) [order 1] : [!IsNewCtrl_Voltage()]
  Current -> (junction 336) [order 2] : [!IsNewCtrl_Idle() && !IsNewCtrl_Position()]
  (junction 336) -> Current [order 2]
  (junction 336) -> (junction 346) [order 1] : [!IsNewCtrl_Current()]
  (junction 337) -> Current : {newSetpoint=ControlOutputs.Iq_fbk.current;}
  (junction 338) -> (junction 337) [order 1] : [IsNewCtrl_Current()]
  HWFault -> (junction 329) [order 2] : [!isInFault && IsNewCtrl_Idle()]
  (junction 347) -> (junction 338) [order 2]
  Current -> (junction 340) [order 1] : [isInFault || isfaultButtonPressedEvent]
  (junction 340) -> (junction 330)
  (junction 330) -> (junction 189)
  (junction 236) -> HWFault
  (junction 339) -> Voltage [order 1] : [IsNewCtrl_Voltage()]{newSetpoint=0; }
  (junction 339) -> (junction 186) [order 2]
  (junction 341) -> (junction 342) [order 1] : [IsNewCtrl_Voltage()]
  (junction 342) -> Voltage : {newSetpoint=ControlOutputs.Vq;}
  (junction 343) -> Voltage [order 2]
  (junction 341) -> (junction 184) [order 2]
  (junction 344) -> (junction 342)
  Voltage -> (junction 343) [order 3]
  (junction 346) -> (junction 344) [order 1] : [IsNewCtrl_Voltage()]
  (junction 346) -> (junction 185) [order 2]
  (junction 345) -> Voltage : {newSetpoint=ControlOutputs.Vq;}
  (junction 347) -> (junction 345) [order 1] : [IsNewCtrl_Voltage()]
  Voltage -> (junction 188) [order 2] : [IsNewCtrl_Velocity()]
  (junction 239) -> (junction 347) [order 1] : [!IsNewCtrl_Velocity()]
  (junction 188) -> Voltage [order 2]
  (junction 188) -> (junction 234) [order 1] : [!IsNewCtrl_Voltage()]
  Voltage -> (junction 187) [order 1] : [isInFault || isfaultButtonPressedEvent]
  (junction 187) -> (junction 189)
  (junction 189) -> (junction 235)
  (junction 186) -> Velocity : [IsNewCtrl_Velocity()]
  (junction 184) -> Velocity : [IsNewCtrl_Velocity()]
  (junction 185) -> Velocity : [IsNewCtrl_Velocity()]
  (junction 239) -> Velocity [order 2]
  (junction 234) -> Velocity : [IsNewCtrl_Velocity()]
  Velocity -> (junction 239) [order 2]
  Velocity -> (junction 240) [order 1] : [isInFault || isfaultButtonPressedEvent]
  (junction 240) -> (junction 235)
  (junction 235) -> (junction 237)
  (junction 237) -> (junction 241) [order 2] : [isfaultButtonPressedEvent]
  (junction 237) -> (junction 236) [order 1] : [isInFault]
  data: isSet function_output boolean; boardIsOK function_output boolean; out function_output boolean; out function_output boolean; out function_output boolean; out function_output boolean; out function_output boolean; boardSt input; areLimitsSet input; requiredControlMode input Enum: ControlModes; SensorsData input; ControlOutputs input; newSetpoint output single; controlModeDefined output Enum: ControlModes; isfaultButtonPressedEvent input boolean; isInFault input boolean
  events: setSetpointEvent_controlModeHandler output FUNCTION_CALL_EVENT
  function isSet = isConfigurationSet:
    | function isSet = isConfigurationSet
    | 
    | % TODO: Add more conditions as more CAN packets are processed.
    | isSet = areLimitsSet; % && IsVoltageLimitSet && IsTemperatureLimitSet;
    | %isSet = isSet && a;
    | end
  function boardIsOK=IsBoardReady:
    | function boardIsOK=IsBoardReady
    |  
    | boardIsOK = (boardSt==BoardState.Configured);
    | 
    | end
  function out=IsNewCtrl_Idle:
    | function out=IsNewCtrl_Idle
    | if(requiredControlMode==ControlModes.Idle)
    |     out=true;
    | else
    |     out=false;
    | end
  function out=IsNewCtrl_Position:
    | function out=IsNewCtrl_Position
    | if(requiredControlMode==ControlModes.Position) 
    |     out=true;
    | else
    |     out=false;
    | end
  function out=IsNewCtrl_Current:
    | function out=IsNewCtrl_Current
    | if(requiredControlMode==ControlModes.Current)
    |     out=true;
    | else
    |     out=false;
    | end
  function out=IsNewCtrl_Velocity:
    | function out=IsNewCtrl_Velocity
    | if(requiredControlMode==ControlModes.Velocity)
    |     out=true;
    | else
    |     out=false;
    | end
  function out=IsNewCtrl_Voltage:
    | function out=IsNewCtrl_Voltage
    | if(requiredControlMode==ControlModes.Voltage)
    |     out=true;
    | else
    |     out=false;
    | end
